simulink model "L2_schema"  (R2026b)
settings: Solver=VariableStepAuto  StopTime=3
settings Model: Creator=oksid  LastModifiedBy=oksid

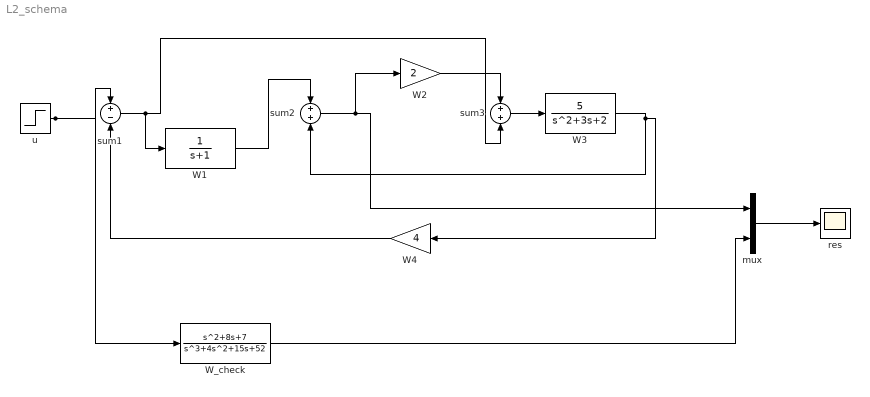
== system L2_schema ==
  W1 : TransferFcn  Denominator=[1 1]
  W2 : Gain  Gain=2
  W3 : TransferFcn  Numerator=[5]  Denominator=[1 3 2]
  W4 : Gain  Gain=4
  W_check : TransferFcn  Numerator=[1 8 7]  Denominator=[1 4 15 52]
  mux : Mux  Inputs=2
  res : Scope
  sum1 : Sum  Inputs=+-
  sum2 : Sum
  sum3 : Sum
  u : Step  SampleTime=0
  wires:
  u/1 -> sum1/1, W_check/1
  sum1/1 -> W1/1, sum3/2
  W1/1 -> sum2/1
  sum2/1 -> W2/1, mux/1
  W2/1 -> sum3/1
  sum3/1 -> W3/1
  W3/1 -> sum2/2, W4/1
  W4/1 -> sum1/2
  W_check/1 -> mux/2
  mux/1 -> res/1
